simulink model "MMC_Rectifier_NLM_2018"  (R2023b)
settings: Solver=ode23t  StartTime=0.0  StopTime=3  RelTol=1e-3
libraries: spsIGBTDiodeLib x216, spsSeriesRLCBranchLib x117, spsVoltageMeasurementLib x110, spsCurrentMeasurementLib x7, slpidlib x6, spsThreePhaseVIMeasurementLib x2, spsGroundLib x1, spsPower3phInstantaneousLib x1, spsThreePhaseProgrammableVoltageSourceLib x1, spsThreePhaseSeriesRLCBranchLib x1, spspowerguiLib x1
(part 1 of 5)
settings Model: Creator=Administrator  LastModifiedBy=Qu
settings SolverCC: AlgebraicLoopSolver=TrustRegion
settings DataIOCC: ReturnWorkspaceOutputs=off
settings DebuggingCC: ArithmeticOperatorsInVariantConditions=warning
settings SFSimCC: CustomCodeUndefinedFunction=UseInterfaceOnly

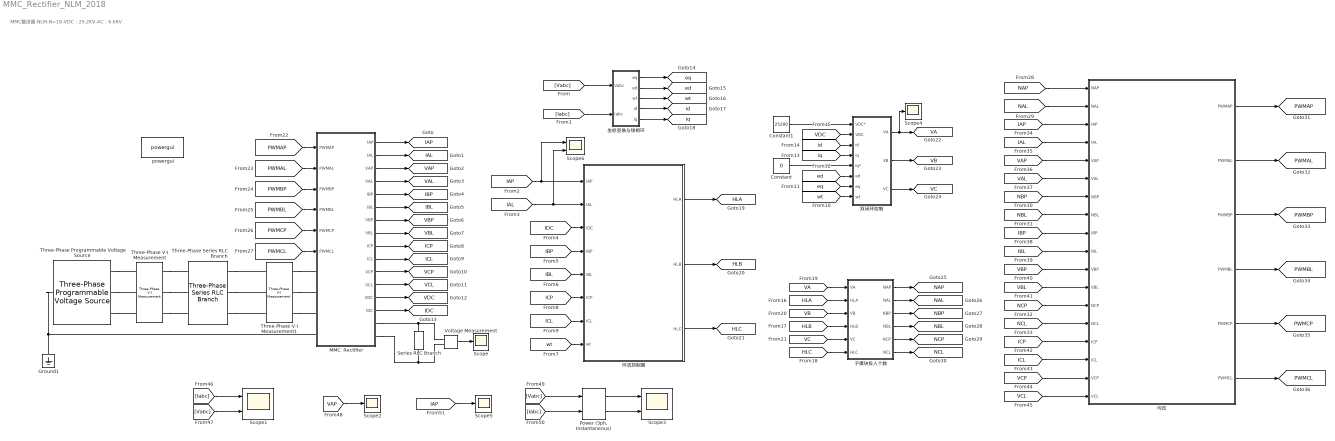
== system MMC_Rectifier_NLM_2018 ==
  note: MMC整流器-NLM-N=18-VDC：25.2KV-AC：6.6KV
  Constant : Constant  Value=0
  Constant1 : Constant  Value=25200
  Ground1 : spsGroundLib/Ground  LConnTagsString=a
  MMC  Rectifier : Subsystem  mask{C0=1.5e-3, V0=1400, C1=1.2e-3, R1=1e-6, L0=0.0577}
      mask prompts: C0 "子模块旁路电容C0"; V0 "子模块电容初始电压V0"; C1 "直流电容C1"; R1 "直流电阻R1"; L0 "桥臂电感L0"
      mask DialogControl ParameterGroupVar Prompt: 参数
  "Power (3ph, Instantaneous)" : spsPower3phInstantaneousLib/Power (3ph, Instantaneous)
  Scope{,2,4..5} (4 alike) : Scope
  Scope1 : Scope  NumInputPorts=2
  Scope3 : Scope  NumInputPorts=2
  Scope6 : Scope  NumInputPorts=2
  Series RLC Branch : spsSeriesRLCBranchLib/Series RLC Branch  LConnTagsString=__new0  RConnTagsString=__new0  BranchType=R  Resistance=200  Inductance=1e-3  SetiL0=off  InitialCurrent=0  Capacitance=1e-6  Setx0=off  InitialVoltage=0  Measurements=None
  Three-Phase Programmable Voltage Source : spsThreePhaseProgrammableVoltageSourceLib/Three-Phase Programmable Voltage Source  PositiveSequence="[6600  0 50]"  VariationEntity=None  VariationType=Table of time-amplitude pairs  VariationTypeAlt=Step  VariationStep=0.5  VariationRate=10  VariationMagnitude=0.3  VariationFrequency=2  VariationTiming=[1 2]  VariationPhaseA=off  Amplitudes=[1 0.8 1.2 1.0]  TimeValues=[0 0.1 0.15 0.2]  HarmonicGeneration=off  HarmonicA=[3 0.2 -25 0]  HarmonicB=[2 0.15 35 2]  Timing="[0.05  3]"  BusType=swing  Pref=0  Qref=0  Qmin=-inf  Qmax=inf
  Three-Phase Series RLC Branch : spsThreePhaseSeriesRLCBranchLib/Three-Phase Series RLC Branch  LConnTagsString=A|B|C  RConnTagsString=A|B|C  BranchType=RL  Resistance=0.5929  Inductance=1e-3  Capacitance=1e-6  Measurements=None
  Three-Phase V-I Measurement : spsThreePhaseVIMeasurementLib/Three-Phase V-I Measurement  VoltageMeasurement=phase-to-ground  SetLabelV=on  LabelV=Vabc  Vpu=off  VpuLL=off  CurrentMeasurement=yes  SetLabelI=on  LabelI=Iabc  Ipu=off  Pbase=100e6  Vbase=500e3  OutputType=Complex  PhasorSimulation=off  PSBequivalent=0
  Three-Phase V-I Measurement1 : spsThreePhaseVIMeasurementLib/Three-Phase V-I Measurement  VoltageMeasurement=phase-to-ground  SetLabelV=on  LabelV=Vin  Vpu=off  VpuLL=off  CurrentMeasurement=yes  SetLabelI=on  LabelI=Iin  Ipu=off  Pbase=100e6  Vbase=500e3  OutputType=Complex  PhasorSimulation=off  PSBequivalent=0
  Voltage Measurement : spsVoltageMeasurementLib/Voltage Measurement  PhasorSimulation=off  OutputType=Complex  PSBequivalent=0
  powergui : spspowerguiLib/powergui  Priority=1  SimulationMode=Discrete  SampleTime=5e-5  frequency=60  Iterations=50  frequencyindice=50  Pbase=100e6  ErrMax=1e-4  UnitsV=kV  UnitsW=MW  buscounter=0  FunctionMessages=off  echomessages=off  EnableUseOfTLC=off  CurrentSourceSwitches=off  DisableSnubberDevices=off  DisableRonSwitches=off  DisableVfSwitches=off  DisplayEquations=off  AutomaticDiscreteSolvers=off  SolverType=Tustin/Backward Euler (TBE)  Interpol=off  ExternalGateDelay=off  methode=off  Ts=100  x0status=blocks  SPID=on  SwTol=0  HookPort=off  NonlinearTolerance=1e-4  nMaxIteration=100  ContinueOnMaxIteration=off  RestoreLinks=warning  ResistiveCurrentMeasurement=off  Frange=[0:2:500]  Ylog=off  Xlog=on  ShowGrid=off  save=off  variable=ZData  structure=0  ZoomFFT=off  StartTime=0.0  cycles=1  DisplayStyle=1  fundamental=60  FreqAxis=off  MaxFrequency=1000  frequencyindicesteady=1  RmsSteady=1  display=off
  双闭环控制 : Subsystem  mask{KP1=0.024467, KI1=0.319, KP2=11.712, KI2=117.263, wL=100*pi*(1e-3+0.0577/2)}
      mask prompts: KP1 "电压外环KP1"; KI1 "电压外环KI1"; KP2 "电流内环KP2"; KI2 "电流内环KI2"; wL "耦合量"
      mask DialogControl ParameterGroupVar Prompt: 参数
  均压 : Subsystem
  坐标变换与锁相环 : Subsystem
  子模块投入个数 : Subsystem  mask{N=18}
      mask prompts: N "子模块个数N"
      mask DialogControl ParameterGroupVar Prompt: 参数
  环流抑制器 : Subsystem  mask{KP=39.04267, KI=117.1793, wL0=100*pi*0.0577}
      mask prompts: KP "环流抑制KP"; KI "环流抑制KI"; wL0 "耦合量wL0"
      mask DialogControl ParameterGroupVar Prompt: 参数
  tag scope: HLA=global, HLB=global, HLC=global, IAL=global, IAP=global, IBL=global, IBP=global, ICL=global, ICP=global, IDC=global, NAL=global, NAP=global, NBL=global, NBP=global, NCL=global, NCP=global, PWMAL=global, PWMAP=global, PWMBL=global, PWMBP=global, PWMCL=global, PWMCP=global, VA=global, VAL=global, VAP=global, VB=global, VBL=global, VBP=global, VC=global, VCL=global, VCP=global, VDC=global, ed=global, eq=global, id=global, iq=global, wt=global
  wires:
  Voltage Measurement/1 -> Scope/1
  MMC  Rectifier/1(IAP) -> [IAP]
  MMC  Rectifier/2(IAL) -> [IAL]
  MMC  Rectifier/3(VAP) -> [VAP]
  MMC  Rectifier/4(VAL) -> [VAL]
  MMC  Rectifier/12(VCL) -> [VCL]
  MMC  Rectifier/11(VCP) -> [VCP]
  MMC  Rectifier/10(ICL) -> [ICL]
  MMC  Rectifier/9(ICP) -> [ICP]
  MMC  Rectifier/8(VBL) -> [VBL]
  MMC  Rectifier/7(VBP) -> [VBP]
  MMC  Rectifier/6(IBL) -> [IBL]
  MMC  Rectifier/5(IBP) -> [IBP]
  MMC  Rectifier/13(VDC) -> [VDC]
  MMC  Rectifier/14(IDC) -> [IDC]
  [Vabc] -> 坐标变换与锁相环/1(Vabc)
  [Iabc] -> 坐标变换与锁相环/2(Iabc)
  坐标变换与锁相环/1(eq) -> [eq]
  坐标变换与锁相环/2(ed) -> [ed]
  坐标变换与锁相环/3(wt) -> [wt]
  坐标变换与锁相环/5(iq) -> [iq]
  坐标变换与锁相环/4(id) -> [id]
  [IAP] -> Scope6/1, 环流抑制器/1(IAP)
  [IAL] -> Scope6/2, 环流抑制器/2(IAL)
  [wt] -> 环流抑制器/8(wt)
  [IDC] -> 环流抑制器/3(IDC)
  [IBP] -> 环流抑制器/4(IBP)
  [IBL] -> 环流抑制器/5(IBL)
  [ICP] -> 环流抑制器/6(ICP)
  [ICL] -> 环流抑制器/7(ICL)
  环流抑制器/2(HLB) -> [HLB]
  环流抑制器/1(HLA) -> [HLA]
  环流抑制器/3(HLC) -> [HLC]
  [wt] -> 双闭环控制/8(wt)
  [eq] -> 双闭环控制/7(eq)
  [ed] -> 双闭环控制/6(ed)
  Constant/1 -> 双闭环控制/5(iq*)
  [id] -> 双闭环控制/3(id)
  [iq] -> 双闭环控制/4(iq)
  [VDC] -> 双闭环控制/2(VDC)
  Constant1/1 -> 双闭环控制/1(VDC*)
  双闭环控制/1(VA) -> Scope4/1, [VA]
  双闭环控制/2(VB) -> [VB]
  双闭环控制/3(VC) -> [VC]
  子模块投入个数/1(NAP) -> [NAP]
  子模块投入个数/2(NAL) -> [NAL]
  子模块投入个数/3(NBP) -> [NBP]
  子模块投入个数/4(NBL) -> [NBL]
  子模块投入个数/5(NCP) -> [NCP]
  子模块投入个数/6(NCL) -> [NCL]
  [HLB] -> 子模块投入个数/4(HLB)
  [HLA] -> 子模块投入个数/2(HLA)
  [HLC] -> 子模块投入个数/6(HLC)
  [VC] -> 子模块投入个数/5(VC)
  [VB] -> 子模块投入个数/3(VB)
  [VA] -> 子模块投入个数/1(VA)
  均压/1(PWMAP) -> [PWMAP]
  均压/2(PWMAL) -> [PWMAL]
  均压/3(PWMBP) -> [PWMBP]
  均压/4(PWMBL) -> [PWMBL]
  均压/5(PWMCP) -> [PWMCP]
  均压/6(PWMCL) -> [PWMCL]
  [PWMBP] -> MMC  Rectifier/3(PWMBP)
  [PWMBL] -> MMC  Rectifier/4(PWMBL)
  [PWMAL] -> MMC  Rectifier/2(PWMAL)
  [PWMAP] -> MMC  Rectifier/1(PWMAP)
  [PWMCP] -> MMC  Rectifier/5(PWMCP)
  [PWMCL] -> MMC  Rectifier/6(PWMCL)
  [NAP] -> 均压/1(NAP)
  [NAL] -> 均压/2(NAL)
  [NBP] -> 均压/7(NBP)
  [NBL] -> 均压/8(NBL)
  [NCP] -> 均压/13(NCP)
  [NCL] -> 均压/14(NCL)
  [IAP] -> 均压/3(IAP)
  [IAL] -> 均压/4(IAL)
  [VAL] -> 均压/6(VAL)
  [VAP] -> 均压/5(VAP)
  [IBP] -> 均压/9(IBP)
  [IBL] -> 均压/10(IBL)
  [VBP] -> 均压/11(VBP)
  [VBL] -> 均压/12(VBL)
  [VCP] -> 均压/17(VCP)
  [ICL] -> 均压/16(ICL)
  [ICP] -> 均压/15(ICP)
  [VCL] -> 均压/18(VCL)
  [Iabc] -> Scope1/1
  [Vabc] -> Scope1/2
  [VAP] -> Scope2/1
  [Vabc] -> "Power (3ph, Instantaneous)"/1
  [Iabc] -> "Power (3ph, Instantaneous)"/2
  "Power (3ph, Instantaneous)"/1 -> Scope3/1
  "Power (3ph, Instantaneous)"/2 -> Scope3/2
  [IAP] -> Scope5/1
  connections:
  Three-Phase Programmable Voltage Source/LConn1 -- MMC  Rectifier/LConn4 -- Ground1/LConn1
  Three-Phase Programmable Voltage Source/RConn1 -- Three-Phase V-I Measurement/LConn1
  Three-Phase Programmable Voltage Source/RConn2 -- Three-Phase V-I Measurement/LConn2
  Three-Phase Programmable Voltage Source/RConn3 -- Three-Phase V-I Measurement/LConn3
  Three-Phase V-I Measurement/RConn1 -- Three-Phase Series RLC Branch/LConn1
  Three-Phase V-I Measurement/RConn2 -- Three-Phase Series RLC Branch/LConn2
  Three-Phase V-I Measurement/RConn3 -- Three-Phase Series RLC Branch/LConn3
  Three-Phase Series RLC Branch/RConn1 -- Three-Phase V-I Measurement1/LConn1
  Three-Phase Series RLC Branch/RConn2 -- Three-Phase V-I Measurement1/LConn2
  Three-Phase Series RLC Branch/RConn3 -- Three-Phase V-I Measurement1/LConn3
  Three-Phase V-I Measurement1/RConn1 -- MMC  Rectifier/LConn1
  Three-Phase V-I Measurement1/RConn2 -- MMC  Rectifier/LConn2
  Three-Phase V-I Measurement1/RConn3 -- MMC  Rectifier/LConn3
  MMC  Rectifier/RConn1 -- Voltage Measurement/LConn1 -- Series RLC Branch/LConn1
  MMC  Rectifier/RConn2 -- Voltage Measurement/LConn2 -- Series RLC Branch/RConn1

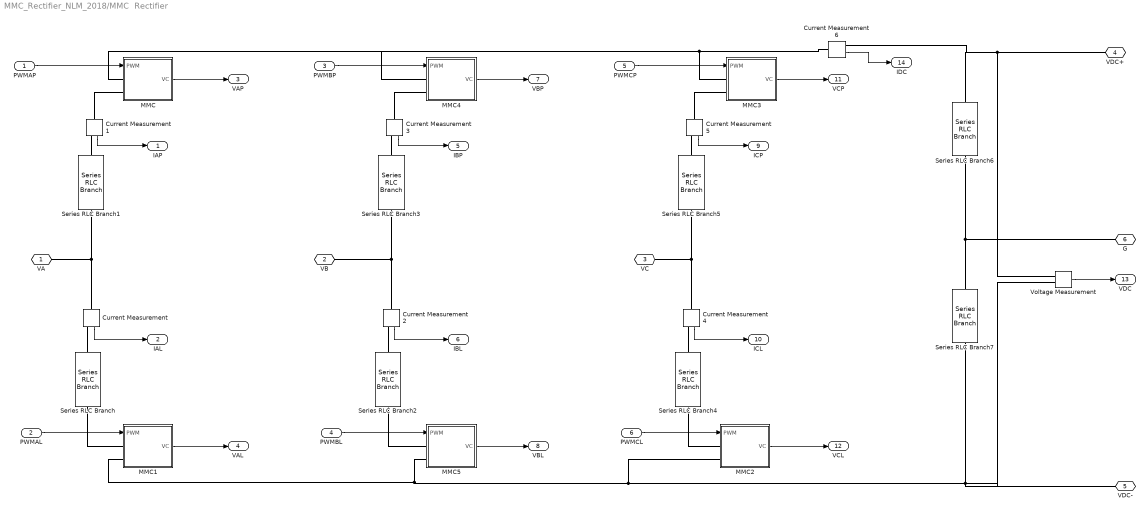
== system MMC_Rectifier_NLM_2018/MMC  Rectifier ==
  PWMAP : Inport
  PWMAL : Inport  Port=2
  PWMBP : Inport  Port=3
  PWMBL : Inport  Port=4
  PWMCP : Inport  Port=5
  PWMCL : Inport  Port=6
  Current Measurement{,1..6} (7 alike) : spsCurrentMeasurementLib/Current Measurement  PhasorSimulation=off  OutputType=Complex  PSBequivalent=0
  MMC : Subsystem
  MMC1 : Subsystem
  MMC2 : Subsystem
  MMC3 : Subsystem
  MMC4 : Subsystem
  MMC5 : Subsystem
  Series RLC Branch{,1..5} (6 alike) : spsSeriesRLCBranchLib/Series RLC Branch  LConnTagsString=__new0  RConnTagsString=__new0  BranchType=L  Resistance=1  Inductance=L0  SetiL0=off  InitialCurrent=0  Capacitance=1e-6  Setx0=off  InitialVoltage=0  Measurements=None
  Series RLC Branch6 : spsSeriesRLCBranchLib/Series RLC Branch  LConnTagsString=__new0  RConnTagsString=__new0  BranchType=RC  Resistance=R1  Inductance=L0  SetiL0=off  InitialCurrent=0  Capacitance=2*C1  Setx0=off  InitialVoltage=3000  Measurements=None
  Series RLC Branch7 : spsSeriesRLCBranchLib/Series RLC Branch  LConnTagsString=__new0  RConnTagsString=__new0  BranchType=RC  Resistance=R1  Inductance=L0  SetiL0=off  InitialCurrent=0  Capacitance=2*C1  Setx0=off  InitialVoltage=3000  Measurements=None
  Voltage Measurement : spsVoltageMeasurementLib/Voltage Measurement  PhasorSimulation=off  OutputType=Complex  PSBequivalent=0
  VA : PMIOPort  Side=Left
  VB : PMIOPort  Port=2  Side=Left
  VC : PMIOPort  Port=3  Side=Left
  VDC+ : PMIOPort  Port=4  Side=Right
  VDC- : PMIOPort  Port=5  Side=Right
  G : PMIOPort  Port=6  Side=Left
  IAP : Outport
  IAL : Outport  Port=2
  VAP : Outport  Port=3
  VAL : Outport  Port=4
  IBP : Outport  Port=5
  IBL : Outport  Port=6
  VBP : Outport  Port=7
  VBL : Outport  Port=8
  ICP : Outport  Port=9
  ICL : Outport  Port=10
  VCP : Outport  Port=11
  VCL : Outport  Port=12
  VDC : Outport  Port=13
  IDC : Outport  Port=14
  wires:
  MMC4/1(VC) -> VBP/1
  Current Measurement1/1 -> IAP/1
  Voltage Measurement/1 -> VDC/1
  PWMAL/1 -> MMC1/1(PWM)
  MMC2/1(VC) -> VCL/1
  MMC/1(VC) -> VAP/1
  MMC1/1(VC) -> VAL/1
  Current Measurement/1 -> IAL/1
  Current Measurement4/1 -> ICL/1
  MMC3/1(VC) -> VCP/1
  MMC5/1(VC) -> VBL/1
  PWMBL/1 -> MMC5/1(PWM)
  PWMBP/1 -> MMC4/1(PWM)
  Current Measurement2/1 -> IBL/1
  Current Measurement3/1 -> IBP/1
  PWMAP/1 -> MMC/1(PWM)
  Current Measurement5/1 -> ICP/1
  PWMCP/1 -> MMC3/1(PWM)
  PWMCL/1 -> MMC2/1(PWM)
  Current Measurement6/1 -> IDC/1
  connections:
  MMC5/LConn1 -- Series RLC Branch2/RConn1
  Series RLC Branch3/RConn1 -- VB/RConn1 -- Current Measurement2/LConn1
  Current Measurement2/RConn1 -- Series RLC Branch2/LConn1
  VDC+/RConn1 -- Current Measurement6/RConn1 -- Series RLC Branch6/LConn1 -- Voltage Measurement/LConn1
  MMC1/LConn1 -- Series RLC Branch/RConn1
  VDC-/RConn1 -- Voltage Measurement/LConn2 -- Series RLC Branch7/RConn1 -- MMC2/LConn2 -- MMC5/LConn2 -- MMC1/LConn2
  Current Measurement3/RConn1 -- Series RLC Branch3/LConn1
  Series RLC Branch5/RConn1 -- VC/RConn1 -- Current Measurement4/LConn1
  Current Measurement5/RConn1 -- Series RLC Branch5/LConn1
  Series RLC Branch1/RConn1 -- VA/RConn1 -- Current Measurement/LConn1
  Current Measurement/RConn1 -- Series RLC Branch/LConn1
  MMC/LConn2 -- Current Measurement1/LConn1
  Current Measurement1/RConn1 -- Series RLC Branch1/LConn1
  MMC4/LConn2 -- Current Measurement3/LConn1
  Current Measurement4/RConn1 -- Series RLC Branch4/LConn1
  MMC2/LConn1 -- Series RLC Branch4/RConn1
  Series RLC Branch6/RConn1 -- G/RConn1 -- Series RLC Branch7/LConn1
  MMC4/LConn1 -- MMC/LConn1 -- MMC3/LConn1 -- Current Measurement6/LConn1
  MMC3/LConn2 -- Current Measurement5/LConn1

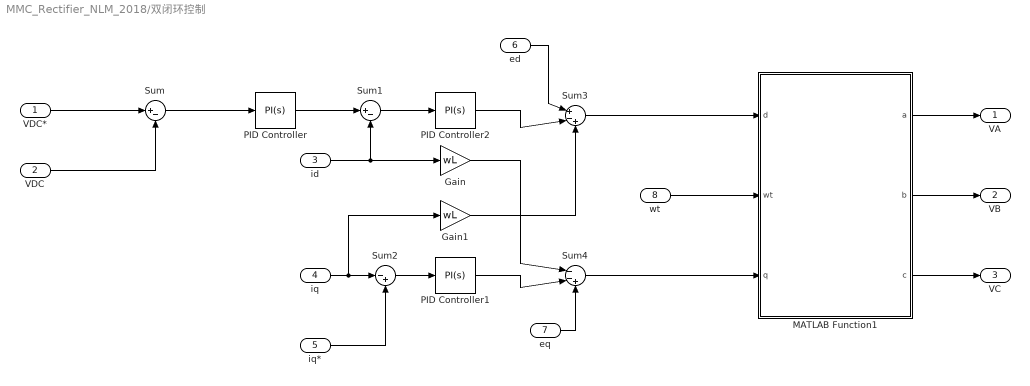
== system MMC_Rectifier_NLM_2018/双闭环控制 ==
  VDC* : Inport
  VDC : Inport  Port=2
  id : Inport  Port=3
  iq : Inport  Port=4
  iq* : Inport  Port=5
  ed : Inport  Port=6
  eq : Inport  Port=7
  wt : Inport  Port=8
  Gain : Gain  Gain=wL
  Gain1 : Gain  Gain=wL
  MATLAB Function1 : MATLAB Function  TreatAsAtomicUnit=on
  PID Controller : slpidlib/PID Controller  Controller=PI  Form=Parallel  TimeDomain=Continuous-time  UseExternalTs=off  SampleTime=-1  IntegratorMethod=Forward Euler  FilterMethod=Forward Euler  ControllerParametersSource=internal  P=KP1  I=KI1  UseKiTs=off  D=0  N=100  UseFilter=on  TunerSelectOption=Transfer Function Based (PID Tuner App)  InitialConditionSource=internal  InitialConditionForIntegrator=0  InitialConditionForFilter=0  DifferentiatorICPrevScaledInput=0  ExternalReset=none  TrackingMode=off  Kt=1  LimitOutput=off  SatLimitsSource=internal  UpperSaturationLimit=inf  LowerSaturationLimit=-inf  LinearizeAsGain=on  AntiWindupMode=none  Kb=1  LimitIntegrator=off  UpperIntegratorSaturationLimit=inf  LowerIntegratorSaturationLimit=-inf  POutMin=[]  POutMax=[]  IOutMin=[]  IOutMax=[]  DOutMin=[]  DOutMax=[]  NOutMin=[]  NOutMax=[]  SumOutMin=[]  SumOutMax=[]  SaturationOutMin=[]  SaturationOutMax=[]  PParamMin=[]  PParamMax=[]  IParamMin=[]  IParamMax=[]  DParamMin=[]  DParamMax=[]  NParamMin=[]  NParamMax=[]  KbParamMin=[]  KbParamMax=[]  KtParamMin=[]  KtParamMax=[]  KbOutMin=[]  KbOutMax=[]  KtOutMin=[]  KtOutMax=[]  IntegratorOutMin=[]  IntegratorOutMax=[]  FilterOutMin=[]  FilterOutMax=[]  SumI1OutMin=[]  SumI1OutMax=[]  SumI2OutMin=[]  SumI2OutMax=[]  SumI3OutMin=[]  SumI3OutMax=[]  SumI4OutMin=[]  SumI4OutMax=[]  SumDOutMin=[]  SumDOutMax=[]  DifferentiatorOutMin=[]  DifferentiatorOutMax=[]  FilterDiffOutCoefMin=[]  FilterDiffOutCoefMax=[]  ReciprocalOutMin=[]  ReciprocalOutMax=[]  SumDenOutMin=[]  SumDenOutMax=[]  SumNumOutMin=[]  SumNumOutMax=[]  DivideOutMin=[]  DivideOutMax=[]  UdiffTsProdOutMin=[]  UdiffTsProdOutMax=[]  NTsProdOutMin=[]  NTsProdOutMax=[]  UintegralTsProdOutMin=[]  UintegralTsProdOutMax=[]  UngainTsProdOutMin=[]  UngainTsProdOutMax=[]  ClampingZeroOutDataTypeStr=Inherit: Inherit via back propagation  ClampingZeroOutMin=[]  ClampingZeroOutMax=[]  FilterDenConstantOutDataTypeStr=Inherit: Inherit via back propagation  FilterDenConstantOutMin=[]  FilterDenConstantOutMax=[]  PCopyOutDataTypeStr=Inherit: Inherit via back propagation  PCopyOutMin=[]  PCopyOutMax=[]  NCopyOutDataTypeStr=Inherit: Inherit via back propagation  NCopyOutMin=[]  NCopyOutMax=[]  IntegratorContinuousStateAttributes=''  IntegratorStateMustResolveToSignalObject=off  IntegratorRTWStateStorageClass=Auto  FilterContinuousStateAttributes=''  FilterStateMustResolveToSignalObject=off  FilterRTWStateStorageClass=Auto  ParallelPVariant=InternalParameters  IdealPVariant=Disabled  IVariant=InternalParameters  DVariant=Disabled  IntegratorVariant=Continuous  SatVariant=Disabled  AWVariant=Passthrough  PCopyVariant=Disabled  TRVariant=Disabled  FdbkBlocksVariant=Forward  IdealPFdbkVariant=Disabled  SatFdbkVariant=Disabled  DerivativeFilterVariant=Disabled  NVariant=Disabled  NCopyVariant=Disabled_SignalSpec  FilterICVariant=Disabled  IntegratorICVariant=InternalICs  ExternalResetVariant=Disabled  TRSumVariant=Passthrough  SumFdbkVariant=Disabled  SumVariant=Sum_PI  TsampFilterVariant=InternalTs  TsampNgainVariant=Passthrough  TsampIntegralVariant=Disabled_SignalSpec  ExternalSaturationOutDataTypeStr=Inherit: Same as second input
  PID Controller1 : slpidlib/PID Controller  Controller=PI  Form=Parallel  TimeDomain=Continuous-time  UseExternalTs=off  SampleTime=-1  IntegratorMethod=Forward Euler  FilterMethod=Forward Euler  ControllerParametersSource=internal  P=KP2  I=KI2  UseKiTs=off  D=0  N=100  UseFilter=on  TunerSelectOption=Transfer Function Based (PID Tuner App)  InitialConditionSource=internal  InitialConditionForIntegrator=0  InitialConditionForFilter=0  DifferentiatorICPrevScaledInput=0  ExternalReset=none  TrackingMode=off  Kt=1  LimitOutput=off  SatLimitsSource=internal  UpperSaturationLimit=inf  LowerSaturationLimit=-inf  LinearizeAsGain=on  AntiWindupMode=none  Kb=1  LimitIntegrator=off  UpperIntegratorSaturationLimit=inf  LowerIntegratorSaturationLimit=-inf  POutMin=[]  POutMax=[]  IOutMin=[]  IOutMax=[]  DOutMin=[]  DOutMax=[]  NOutMin=[]  NOutMax=[]  SumOutMin=[]  SumOutMax=[]  SaturationOutMin=[]  SaturationOutMax=[]  PParamMin=[]  PParamMax=[]  IParamMin=[]  IParamMax=[]  DParamMin=[]  DParamMax=[]  NParamMin=[]  NParamMax=[]  KbParamMin=[]  KbParamMax=[]  KtParamMin=[]  KtParamMax=[]  KbOutMin=[]  KbOutMax=[]  KtOutMin=[]  KtOutMax=[]  IntegratorOutMin=[]  IntegratorOutMax=[]  FilterOutMin=[]  FilterOutMax=[]  SumI1OutMin=[]  SumI1OutMax=[]  SumI2OutMin=[]  SumI2OutMax=[]  SumI3OutMin=[]  SumI3OutMax=[]  SumI4OutMin=[]  SumI4OutMax=[]  SumDOutMin=[]  SumDOutMax=[]  DifferentiatorOutMin=[]  DifferentiatorOutMax=[]  FilterDiffOutCoefMin=[]  FilterDiffOutCoefMax=[]  ReciprocalOutMin=[]  ReciprocalOutMax=[]  SumDenOutMin=[]  SumDenOutMax=[]  SumNumOutMin=[]  SumNumOutMax=[]  DivideOutMin=[]  DivideOutMax=[]  UdiffTsProdOutMin=[]  UdiffTsProdOutMax=[]  NTsProdOutMin=[]  NTsProdOutMax=[]  UintegralTsProdOutMin=[]  UintegralTsProdOutMax=[]  UngainTsProdOutMin=[]  UngainTsProdOutMax=[]  ClampingZeroOutDataTypeStr=Inherit: Inherit via back propagation  ClampingZeroOutMin=[]  ClampingZeroOutMax=[]  FilterDenConstantOutDataTypeStr=Inherit: Inherit via back propagation  FilterDenConstantOutMin=[]  FilterDenConstantOutMax=[]  PCopyOutDataTypeStr=Inherit: Inherit via back propagation  PCopyOutMin=[]  PCopyOutMax=[]  NCopyOutDataTypeStr=Inherit: Inherit via back propagation  NCopyOutMin=[]  NCopyOutMax=[]  IntegratorContinuousStateAttributes=''  IntegratorStateMustResolveToSignalObject=off  IntegratorRTWStateStorageClass=Auto  FilterContinuousStateAttributes=''  FilterStateMustResolveToSignalObject=off  FilterRTWStateStorageClass=Auto  ParallelPVariant=InternalParameters  IdealPVariant=Disabled  IVariant=InternalParameters  DVariant=Disabled  IntegratorVariant=Continuous  SatVariant=Disabled  AWVariant=Passthrough  PCopyVariant=Disabled  TRVariant=Disabled  FdbkBlocksVariant=Forward  IdealPFdbkVariant=Disabled  SatFdbkVariant=Disabled  DerivativeFilterVariant=Disabled  NVariant=Disabled  NCopyVariant=Disabled_SignalSpec  FilterICVariant=Disabled  IntegratorICVariant=InternalICs  ExternalResetVariant=Disabled  TRSumVariant=Passthrough  SumFdbkVariant=Disabled  SumVariant=Sum_PI  TsampFilterVariant=InternalTs  TsampNgainVariant=Passthrough  TsampIntegralVariant=Disabled_SignalSpec  ExternalSaturationOutDataTypeStr=Inherit: Same as second input
  PID Controller2 : slpidlib/PID Controller  Controller=PI  Form=Parallel  TimeDomain=Continuous-time  UseExternalTs=off  SampleTime=-1  IntegratorMethod=Forward Euler  FilterMethod=Forward Euler  ControllerParametersSource=internal  P=KP2  I=KI2  UseKiTs=off  D=0  N=100  UseFilter=on  TunerSelectOption=Transfer Function Based (PID Tuner App)  InitialConditionSource=internal  InitialConditionForIntegrator=0  InitialConditionForFilter=0  DifferentiatorICPrevScaledInput=0  ExternalReset=none  TrackingMode=off  Kt=1  LimitOutput=off  SatLimitsSource=internal  UpperSaturationLimit=inf  LowerSaturationLimit=-inf  LinearizeAsGain=on  AntiWindupMode=none  Kb=1  LimitIntegrator=off  UpperIntegratorSaturationLimit=inf  LowerIntegratorSaturationLimit=-inf  POutMin=[]  POutMax=[]  IOutMin=[]  IOutMax=[]  DOutMin=[]  DOutMax=[]  NOutMin=[]  NOutMax=[]  SumOutMin=[]  SumOutMax=[]  SaturationOutMin=[]  SaturationOutMax=[]  PParamMin=[]  PParamMax=[]  IParamMin=[]  IParamMax=[]  DParamMin=[]  DParamMax=[]  NParamMin=[]  NParamMax=[]  KbParamMin=[]  KbParamMax=[]  KtParamMin=[]  KtParamMax=[]  KbOutMin=[]  KbOutMax=[]  KtOutMin=[]  KtOutMax=[]  IntegratorOutMin=[]  IntegratorOutMax=[]  FilterOutMin=[]  FilterOutMax=[]  SumI1OutMin=[]  SumI1OutMax=[]  SumI2OutMin=[]  SumI2OutMax=[]  SumI3OutMin=[]  SumI3OutMax=[]  SumI4OutMin=[]  SumI4OutMax=[]  SumDOutMin=[]  SumDOutMax=[]  DifferentiatorOutMin=[]  DifferentiatorOutMax=[]  FilterDiffOutCoefMin=[]  FilterDiffOutCoefMax=[]  ReciprocalOutMin=[]  ReciprocalOutMax=[]  SumDenOutMin=[]  SumDenOutMax=[]  SumNumOutMin=[]  SumNumOutMax=[]  DivideOutMin=[]  DivideOutMax=[]  UdiffTsProdOutMin=[]  UdiffTsProdOutMax=[]  NTsProdOutMin=[]  NTsProdOutMax=[]  UintegralTsProdOutMin=[]  UintegralTsProdOutMax=[]  UngainTsProdOutMin=[]  UngainTsProdOutMax=[]  ClampingZeroOutDataTypeStr=Inherit: Inherit via back propagation  ClampingZeroOutMin=[]  ClampingZeroOutMax=[]  FilterDenConstantOutDataTypeStr=Inherit: Inherit via back propagation  FilterDenConstantOutMin=[]  FilterDenConstantOutMax=[]  PCopyOutDataTypeStr=Inherit: Inherit via back propagation  PCopyOutMin=[]  PCopyOutMax=[]  NCopyOutDataTypeStr=Inherit: Inherit via back propagation  NCopyOutMin=[]  NCopyOutMax=[]  IntegratorContinuousStateAttributes=''  IntegratorStateMustResolveToSignalObject=off  IntegratorRTWStateStorageClass=Auto  FilterContinuousStateAttributes=''  FilterStateMustResolveToSignalObject=off  FilterRTWStateStorageClass=Auto  ParallelPVariant=InternalParameters  IdealPVariant=Disabled  IVariant=InternalParameters  DVariant=Disabled  IntegratorVariant=Continuous  SatVariant=Disabled  AWVariant=Passthrough  PCopyVariant=Disabled  TRVariant=Disabled  FdbkBlocksVariant=Forward  IdealPFdbkVariant=Disabled  SatFdbkVariant=Disabled  DerivativeFilterVariant=Disabled  NVariant=Disabled  NCopyVariant=Disabled_SignalSpec  FilterICVariant=Disabled  IntegratorICVariant=InternalICs  ExternalResetVariant=Disabled  TRSumVariant=Passthrough  SumFdbkVariant=Disabled  SumVariant=Sum_PI  TsampFilterVariant=InternalTs  TsampNgainVariant=Passthrough  TsampIntegralVariant=Disabled_SignalSpec  ExternalSaturationOutDataTypeStr=Inherit: Same as second input
  Sum : Sum  Inputs=|+-
  Sum1 : Sum  Inputs=|+-
  Sum2 : Sum  Inputs=|-+
  Sum3 : Sum  Inputs=|+-+
  Sum4 : Sum  Inputs=|--+
  VA : Outport
  VB : Outport  Port=2
  VC : Outport  Port=3
  wires:
  ed/1 -> Sum3/1
  iq*/1 -> Sum2/2
  VDC*/1 -> Sum/1
  VDC/1 -> Sum/2
  iq/1 -> Gain1/1, Sum2/1
  Sum3/1 -> MATLAB Function1/1(d)
  Sum4/1 -> MATLAB Function1/3(q)
  PID Controller1/1 -> Sum4/2
  Sum2/1 -> PID Controller1/1
  MATLAB Function1/1(a) -> VA/1
  id/1 -> Gain/1, Sum1/2
  Sum/1 -> PID Controller/1
  Sum1/1 -> PID Controller2/1
  PID Controller/1 -> Sum1/1
  Gain1/1 -> Sum3/3
  wt/1 -> MATLAB Function1/2(wt)
  MATLAB Function1/3(c) -> VC/1
  PID Controller2/1 -> Sum3/2
  MATLAB Function1/2(b) -> VB/1
  Gain/1 -> Sum4/1
  eq/1 -> Sum4/3

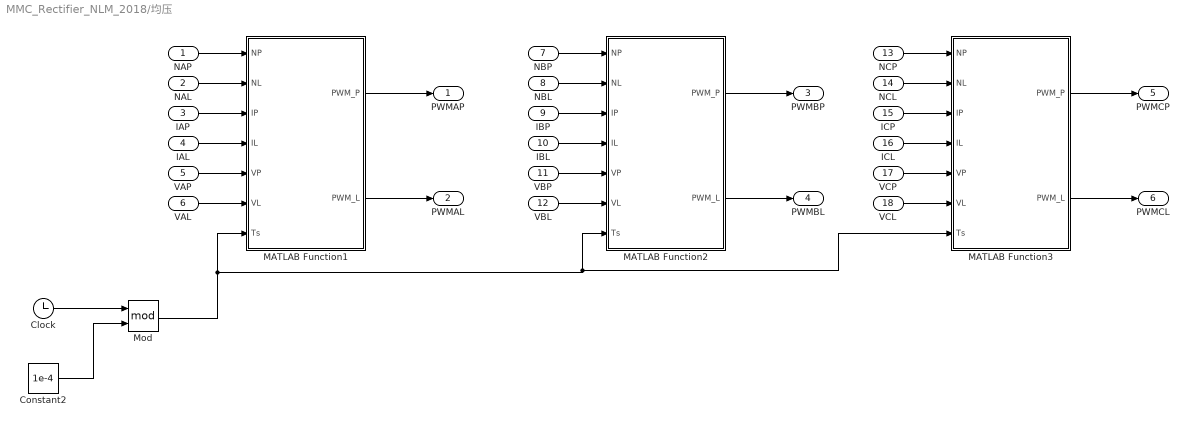
== system MMC_Rectifier_NLM_2018/均压 ==
  NAP : Inport
  NAL : Inport  Port=2
  IAP : Inport  Port=3
  IAL : Inport  Port=4
  VAP : Inport  Port=5
  VAL : Inport  Port=6
  NBP : Inport  Port=7
  NBL : Inport  Port=8
  IBP : Inport  Port=9
  IBL : Inport  Port=10
  VBP : Inport  Port=11
  VBL : Inport  Port=12
  NCP : Inport  Port=13
  NCL : Inport  Port=14
  ICP : Inport  Port=15
  ICL : Inport  Port=16
  VCP : Inport  Port=17
  VCL : Inport  Port=18
  Clock : Clock
  Constant2 : Constant  Value=1e-4
  MATLAB Function1 : MATLAB Function  TreatAsAtomicUnit=on
  MATLAB Function2 : MATLAB Function  TreatAsAtomicUnit=on
  MATLAB Function3 : MATLAB Function  TreatAsAtomicUnit=on
  Mod : Math  Operator=mod  SignedPower=on
  PWMAP : Outport
  PWMAL : Outport  Port=2
  PWMBP : Outport  Port=3
  PWMBL : Outport  Port=4
  PWMCP : Outport  Port=5
  PWMCL : Outport  Port=6
  wires:
  NAL/1 -> MATLAB Function1/2(NL)
  NCP/1 -> MATLAB Function3/1(NP)
  Constant2/1 -> Mod/2
  Mod/1 -> MATLAB Function1/7(Ts), MATLAB Function3/7(Ts), MATLAB Function2/7(Ts)
  VCP/1 -> MATLAB Function3/5(VP)
  MATLAB Function2/2(PWM_L) -> PWMBL/1
  IAP/1 -> MATLAB Function1/3(IP)
  Clock/1 -> Mod/1
  MATLAB Function1/2(PWM_L) -> PWMAL/1
  ICL/1 -> MATLAB Function3/4(IL)
  MATLAB Function1/1(PWM_P) -> PWMAP/1
  VBL/1 -> MATLAB Function2/6(VL)
  IAL/1 -> MATLAB Function1/4(IL)
  MATLAB Function3/2(PWM_L) -> PWMCL/1
  VBP/1 -> MATLAB Function2/5(VP)
  VAL/1 -> MATLAB Function1/6(VL)
  VCL/1 -> MATLAB Function3/6(VL)
  MATLAB Function2/1(PWM_P) -> PWMBP/1
  NBP/1 -> MATLAB Function2/1(NP)
  NBL/1 -> MATLAB Function2/2(NL)
  ICP/1 -> MATLAB Function3/3(IP)
  IBP/1 -> MATLAB Function2/3(IP)
  IBL/1 -> MATLAB Function2/4(IL)
  NAP/1 -> MATLAB Function1/1(NP)
  VAP/1 -> MATLAB Function1/5(VP)
  MATLAB Function3/1(PWM_P) -> PWMCP/1
  NCL/1 -> MATLAB Function3/2(NL)

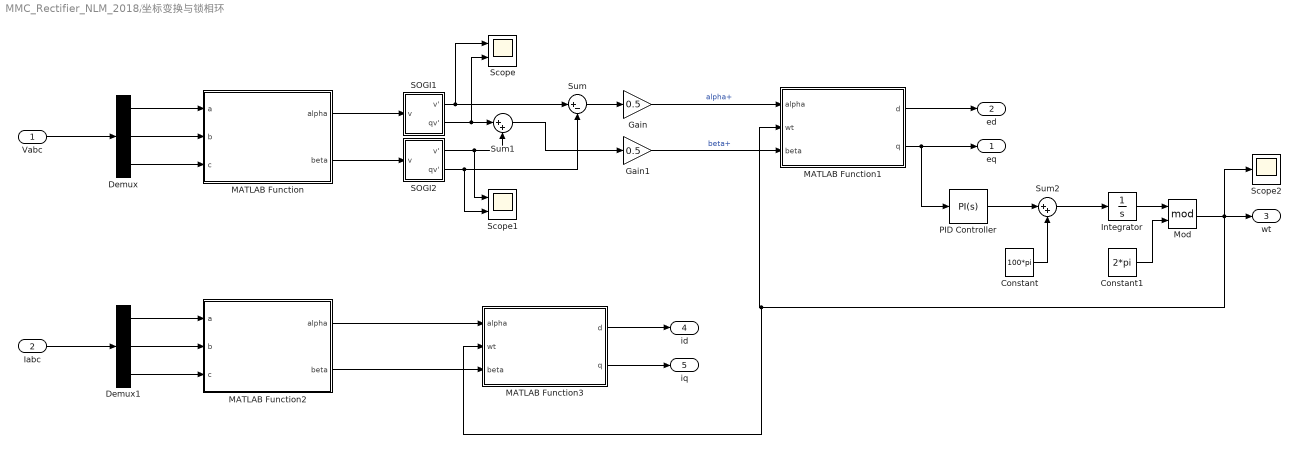
== system MMC_Rectifier_NLM_2018/坐标变换与锁相环 ==
  Vabc : Inport
  Iabc : Inport  Port=2
  Constant : Constant  Value=100*pi
  Constant1 : Constant  Value=2*pi
  Demux : Demux  Outputs=3
  Demux1 : Demux  Outputs=3
  Gain : Gain  Gain=0.5
  Gain1 : Gain  Gain=0.5
  Integrator : Integrator
  MATLAB Function : MATLAB Function  TreatAsAtomicUnit=on
  MATLAB Function1 : MATLAB Function  TreatAsAtomicUnit=on
  MATLAB Function2 : MATLAB Function  TreatAsAtomicUnit=on
  MATLAB Function3 : MATLAB Function  TreatAsAtomicUnit=on
  Mod : Math  Operator=mod  SignedPower=on
  PID Controller : slpidlib/PID Controller  Controller=PI  Form=Parallel  TimeDomain=Continuous-time  UseExternalTs=off  SampleTime=-1  IntegratorMethod=Forward Euler  FilterMethod=Forward Euler  ControllerParametersSource=internal  P=5  I=1/200  UseKiTs=off  D=0  N=100  UseFilter=on  TunerSelectOption=Transfer Function Based (PID Tuner App)  InitialConditionSource=internal  InitialConditionForIntegrator=0  InitialConditionForFilter=0  DifferentiatorICPrevScaledInput=0  ExternalReset=none  TrackingMode=off  Kt=1  LimitOutput=off  SatLimitsSource=internal  UpperSaturationLimit=inf  LowerSaturationLimit=-inf  LinearizeAsGain=on  AntiWindupMode=none  Kb=1  LimitIntegrator=off  UpperIntegratorSaturationLimit=inf  LowerIntegratorSaturationLimit=-inf  POutMin=[]  POutMax=[]  IOutMin=[]  IOutMax=[]  DOutMin=[]  DOutMax=[]  NOutMin=[]  NOutMax=[]  SumOutMin=[]  SumOutMax=[]  SaturationOutMin=[]  SaturationOutMax=[]  PParamMin=[]  PParamMax=[]  IParamMin=[]  IParamMax=[]  DParamMin=[]  DParamMax=[]  NParamMin=[]  NParamMax=[]  KbParamMin=[]  KbParamMax=[]  KtParamMin=[]  KtParamMax=[]  KbOutMin=[]  KbOutMax=[]  KtOutMin=[]  KtOutMax=[]  IntegratorOutMin=[]  IntegratorOutMax=[]  FilterOutMin=[]  FilterOutMax=[]  SumI1OutMin=[]  SumI1OutMax=[]  SumI2OutMin=[]  SumI2OutMax=[]  SumI3OutMin=[]  SumI3OutMax=[]  SumI4OutMin=[]  SumI4OutMax=[]  SumDOutMin=[]  SumDOutMax=[]  DifferentiatorOutMin=[]  DifferentiatorOutMax=[]  FilterDiffOutCoefMin=[]  FilterDiffOutCoefMax=[]  ReciprocalOutMin=[]  ReciprocalOutMax=[]  SumDenOutMin=[]  SumDenOutMax=[]  SumNumOutMin=[]  SumNumOutMax=[]  DivideOutMin=[]  DivideOutMax=[]  UdiffTsProdOutMin=[]  UdiffTsProdOutMax=[]  NTsProdOutMin=[]  NTsProdOutMax=[]  UintegralTsProdOutMin=[]  UintegralTsProdOutMax=[]  UngainTsProdOutMin=[]  UngainTsProdOutMax=[]  ClampingZeroOutDataTypeStr=Inherit: Inherit via back propagation  ClampingZeroOutMin=[]  ClampingZeroOutMax=[]  FilterDenConstantOutDataTypeStr=Inherit: Inherit via back propagation  FilterDenConstantOutMin=[]  FilterDenConstantOutMax=[]  PCopyOutDataTypeStr=Inherit: Inherit via back propagation  PCopyOutMin=[]  PCopyOutMax=[]  NCopyOutDataTypeStr=Inherit: Inherit via back propagation  NCopyOutMin=[]  NCopyOutMax=[]  IntegratorContinuousStateAttributes=''  IntegratorStateMustResolveToSignalObject=off  IntegratorRTWStateStorageClass=Auto  FilterContinuousStateAttributes=''  FilterStateMustResolveToSignalObject=off  FilterRTWStateStorageClass=Auto  ParallelPVariant=InternalParameters  IdealPVariant=Disabled  IVariant=InternalParameters  DVariant=Disabled  IntegratorVariant=Continuous  SatVariant=Disabled  AWVariant=Passthrough  PCopyVariant=Disabled  TRVariant=Disabled  FdbkBlocksVariant=Forward  IdealPFdbkVariant=Disabled  SatFdbkVariant=Disabled  DerivativeFilterVariant=Disabled  NVariant=Disabled  NCopyVariant=Disabled_SignalSpec  FilterICVariant=Disabled  IntegratorICVariant=InternalICs  ExternalResetVariant=Disabled  TRSumVariant=Passthrough  SumFdbkVariant=Disabled  SumVariant=Sum_PI  TsampFilterVariant=InternalTs  TsampNgainVariant=Passthrough  TsampIntegralVariant=Disabled_SignalSpec  ExternalSaturationOutDataTypeStr=Inherit: Same as second input
  SOGI1 : Subsystem
  SOGI2 : Subsystem
  Scope : Scope  NumInputPorts=2
  Scope1 : Scope  NumInputPorts=2
  Scope2 : Scope
  Sum : Sum  Inputs=|+-
  Sum1 : Sum  Inputs=|++
  Sum2 : Sum  Inputs=|++
  eq : Outport
  ed : Outport  Port=2
  wt : Outport  Port=3
  id : Outport  Port=4
  iq : Outport  Port=5
  wires:
  Demux/3 -> MATLAB Function/3(c)
  MATLAB Function1/2(q) -> PID Controller/1, eq/1
  Gain/1 -> MATLAB Function1/1(alpha)  "alpha+"
  Vabc/1 -> Demux/1
  Gain1/1 -> MATLAB Function1/3(beta)  "beta+"
  Demux/2 -> MATLAB Function/2(b)
  Demux/1 -> MATLAB Function/1(a)
  SOGI2/2(qv') -> Scope1/2, Sum/2
  Iabc/1 -> Demux1/1
  Sum1/1 -> Gain1/1
  Demux1/2 -> MATLAB Function2/2(b)
  MATLAB Function/2(beta) -> SOGI2/1(v)
  MATLAB Function2/2(beta) -> MATLAB Function3/3(beta)
  SOGI1/1(v') -> Scope/1, Sum/1
  MATLAB Function/1(alpha) -> SOGI1/1(v)
  SOGI1/2(qv') -> Scope/2, Sum1/1
  Sum/1 -> Gain/1
  SOGI2/1(v') -> Scope1/1, Sum1/2
  MATLAB Function1/1(d) -> ed/1
  Constant/1 -> Sum2/2
  MATLAB Function3/2(q) -> iq/1
  PID Controller/1 -> Sum2/1
  Integrator/1 -> Mod/1
  Demux1/1 -> MATLAB Function2/1(a)
  Demux1/3 -> MATLAB Function2/3(c)
  MATLAB Function2/1(alpha) -> MATLAB Function3/1(alpha)
  Constant1/1 -> Mod/2
  Sum2/1 -> Integrator/1
  MATLAB Function3/1(d) -> id/1
  Mod/1 -> MATLAB Function3/2(wt), MATLAB Function1/2(wt), Scope2/1, wt/1

== system MMC_Rectifier_NLM_2018/子模块投入个数 ==
  VA : Inport
  HLA : Inport  Port=2
  VB : Inport  Port=3
  HLB : Inport  Port=4
  VC : Inport  Port=5
  HLC : Inport  Port=6
  Subsystem : Subsystem
  Subsystem1 : Subsystem
  Subsystem2 : Subsystem
  Subsystem3 : Subsystem
  Subsystem4 : Subsystem
  Subsystem5 : Subsystem
  NAP : Outport
  NAL : Outport  Port=2
  NBP : Outport  Port=3
  NBL : Outport  Port=4
  NCP : Outport  Port=5
  NCL : Outport  Port=6
  wires:
  HLB/1 -> Subsystem3/2(HLB), Subsystem2/2(HLB)
  VB/1 -> Subsystem3/1(VB), Subsystem2/1(VB)
  HLA/1 -> Subsystem1/2(HLA), Subsystem/2(HLA)
  VC/1 -> Subsystem5/1(VC), Subsystem4/1(VC)
  VA/1 -> Subsystem1/1(VA), Subsystem/1(VA)
  Subsystem2/1(NBP) -> NBP/1
  HLC/1 -> Subsystem5/2(HLC), Subsystem4/2(HLC)
  Subsystem/1(NAP) -> NAP/1
  Subsystem3/1(NBL) -> NBL/1
  Subsystem5/1(NCL) -> NCL/1
  Subsystem1/1(NAL) -> NAL/1
  Subsystem4/1(NCP) -> NCP/1

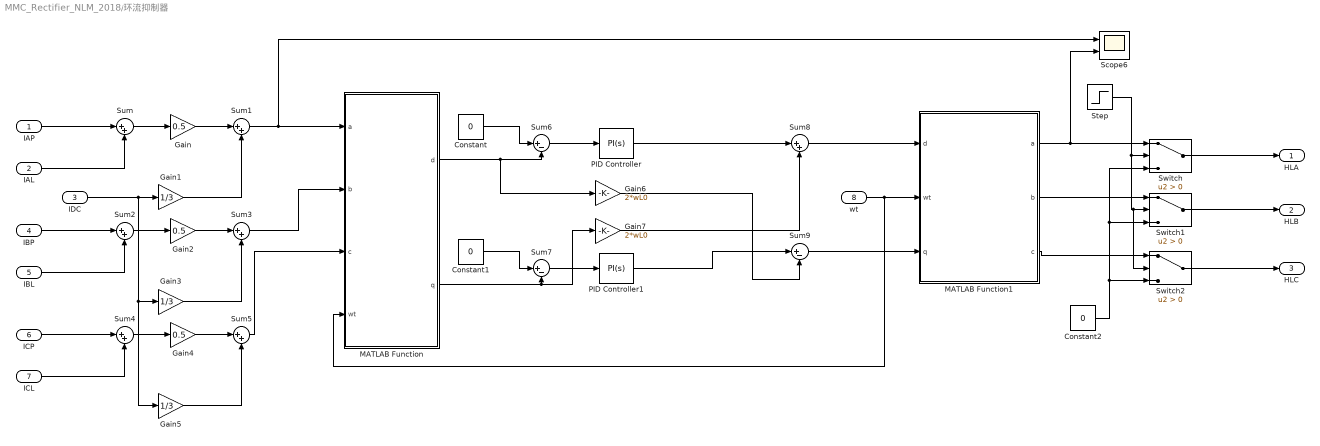
== system MMC_Rectifier_NLM_2018/环流抑制器 ==
  IAP : Inport
  IAL : Inport  Port=2
  IDC : Inport  Port=3
  IBP : Inport  Port=4
  IBL : Inport  Port=5
  ICP : Inport  Port=6
  ICL : Inport  Port=7
  wt : Inport  Port=8
  Constant : Constant  Value=0
  Constant1 : Constant  Value=0
  Constant2 : Constant  Value=0
  Gain : Gain  Gain=0.5
  Gain1 : Gain  Gain=1/3
  Gain2 : Gain  Gain=0.5
  Gain3 : Gain  Gain=1/3
  Gain4 : Gain  Gain=0.5
  Gain5 : Gain  Gain=1/3
  Gain6 : Gain  Gain=2*wL0
  Gain7 : Gain  Gain=2*wL0
  MATLAB Function : MATLAB Function  TreatAsAtomicUnit=on
  MATLAB Function1 : MATLAB Function  TreatAsAtomicUnit=on
  PID Controller : slpidlib/PID Controller  Controller=PI  Form=Parallel  TimeDomain=Continuous-time  UseExternalTs=off  SampleTime=-1  IntegratorMethod=Forward Euler  FilterMethod=Forward Euler  ControllerParametersSource=internal  P=KP  I=KI  UseKiTs=off  D=0  N=100  UseFilter=on  TunerSelectOption=Transfer Function Based (PID Tuner App)  InitialConditionSource=internal  InitialConditionForIntegrator=0  InitialConditionForFilter=0  DifferentiatorICPrevScaledInput=0  ExternalReset=none  TrackingMode=off  Kt=1  LimitOutput=off  SatLimitsSource=internal  UpperSaturationLimit=inf  LowerSaturationLimit=-inf  LinearizeAsGain=on  AntiWindupMode=none  Kb=1  LimitIntegrator=off  UpperIntegratorSaturationLimit=inf  LowerIntegratorSaturationLimit=-inf  POutMin=[]  POutMax=[]  IOutMin=[]  IOutMax=[]  DOutMin=[]  DOutMax=[]  NOutMin=[]  NOutMax=[]  SumOutMin=[]  SumOutMax=[]  SaturationOutMin=[]  SaturationOutMax=[]  PParamMin=[]  PParamMax=[]  IParamMin=[]  IParamMax=[]  DParamMin=[]  DParamMax=[]  NParamMin=[]  NParamMax=[]  KbParamMin=[]  KbParamMax=[]  KtParamMin=[]  KtParamMax=[]  KbOutMin=[]  KbOutMax=[]  KtOutMin=[]  KtOutMax=[]  IntegratorOutMin=[]  IntegratorOutMax=[]  FilterOutMin=[]  FilterOutMax=[]  SumI1OutMin=[]  SumI1OutMax=[]  SumI2OutMin=[]  SumI2OutMax=[]  SumI3OutMin=[]  SumI3OutMax=[]  SumI4OutMin=[]  SumI4OutMax=[]  SumDOutMin=[]  SumDOutMax=[]  DifferentiatorOutMin=[]  DifferentiatorOutMax=[]  FilterDiffOutCoefMin=[]  FilterDiffOutCoefMax=[]  ReciprocalOutMin=[]  ReciprocalOutMax=[]  SumDenOutMin=[]  SumDenOutMax=[]  SumNumOutMin=[]  SumNumOutMax=[]  DivideOutMin=[]  DivideOutMax=[]  UdiffTsProdOutMin=[]  UdiffTsProdOutMax=[]  NTsProdOutMin=[]  NTsProdOutMax=[]  UintegralTsProdOutMin=[]  UintegralTsProdOutMax=[]  UngainTsProdOutMin=[]  UngainTsProdOutMax=[]  ClampingZeroOutDataTypeStr=Inherit: Inherit via back propagation  ClampingZeroOutMin=[]  ClampingZeroOutMax=[]  FilterDenConstantOutDataTypeStr=Inherit: Inherit via back propagation  FilterDenConstantOutMin=[]  FilterDenConstantOutMax=[]  PCopyOutDataTypeStr=Inherit: Inherit via back propagation  PCopyOutMin=[]  PCopyOutMax=[]  NCopyOutDataTypeStr=Inherit: Inherit via back propagation  NCopyOutMin=[]  NCopyOutMax=[]  IntegratorContinuousStateAttributes=''  IntegratorStateMustResolveToSignalObject=off  IntegratorRTWStateStorageClass=Auto  FilterContinuousStateAttributes=''  FilterStateMustResolveToSignalObject=off  FilterRTWStateStorageClass=Auto  ParallelPVariant=InternalParameters  IdealPVariant=Disabled  IVariant=InternalParameters  DVariant=Disabled  IntegratorVariant=Continuous  SatVariant=Disabled  AWVariant=Passthrough  PCopyVariant=Disabled  TRVariant=Disabled  FdbkBlocksVariant=Forward  IdealPFdbkVariant=Disabled  SatFdbkVariant=Disabled  DerivativeFilterVariant=Disabled  NVariant=Disabled  NCopyVariant=Disabled_SignalSpec  FilterICVariant=Disabled  IntegratorICVariant=InternalICs  ExternalResetVariant=Disabled  TRSumVariant=Passthrough  SumFdbkVariant=Disabled  SumVariant=Sum_PI  TsampFilterVariant=InternalTs  TsampNgainVariant=Passthrough  TsampIntegralVariant=Disabled_SignalSpec  ExternalSaturationOutDataTypeStr=Inherit: Same as second input
  PID Controller1 : slpidlib/PID Controller  Controller=PI  Form=Parallel  TimeDomain=Continuous-time  UseExternalTs=off  SampleTime=-1  IntegratorMethod=Forward Euler  FilterMethod=Forward Euler  ControllerParametersSource=internal  P=KP  I=KI  UseKiTs=off  D=0  N=100  UseFilter=on  TunerSelectOption=Transfer Function Based (PID Tuner App)  InitialConditionSource=internal  InitialConditionForIntegrator=0  InitialConditionForFilter=0  DifferentiatorICPrevScaledInput=0  ExternalReset=none  TrackingMode=off  Kt=1  LimitOutput=off  SatLimitsSource=internal  UpperSaturationLimit=inf  LowerSaturationLimit=-inf  LinearizeAsGain=on  AntiWindupMode=none  Kb=1  LimitIntegrator=off  UpperIntegratorSaturationLimit=inf  LowerIntegratorSaturationLimit=-inf  POutMin=[]  POutMax=[]  IOutMin=[]  IOutMax=[]  DOutMin=[]  DOutMax=[]  NOutMin=[]  NOutMax=[]  SumOutMin=[]  SumOutMax=[]  SaturationOutMin=[]  SaturationOutMax=[]  PParamMin=[]  PParamMax=[]  IParamMin=[]  IParamMax=[]  DParamMin=[]  DParamMax=[]  NParamMin=[]  NParamMax=[]  KbParamMin=[]  KbParamMax=[]  KtParamMin=[]  KtParamMax=[]  KbOutMin=[]  KbOutMax=[]  KtOutMin=[]  KtOutMax=[]  IntegratorOutMin=[]  IntegratorOutMax=[]  FilterOutMin=[]  FilterOutMax=[]  SumI1OutMin=[]  SumI1OutMax=[]  SumI2OutMin=[]  SumI2OutMax=[]  SumI3OutMin=[]  SumI3OutMax=[]  SumI4OutMin=[]  SumI4OutMax=[]  SumDOutMin=[]  SumDOutMax=[]  DifferentiatorOutMin=[]  DifferentiatorOutMax=[]  FilterDiffOutCoefMin=[]  FilterDiffOutCoefMax=[]  ReciprocalOutMin=[]  ReciprocalOutMax=[]  SumDenOutMin=[]  SumDenOutMax=[]  SumNumOutMin=[]  SumNumOutMax=[]  DivideOutMin=[]  DivideOutMax=[]  UdiffTsProdOutMin=[]  UdiffTsProdOutMax=[]  NTsProdOutMin=[]  NTsProdOutMax=[]  UintegralTsProdOutMin=[]  UintegralTsProdOutMax=[]  UngainTsProdOutMin=[]  UngainTsProdOutMax=[]  ClampingZeroOutDataTypeStr=Inherit: Inherit via back propagation  ClampingZeroOutMin=[]  ClampingZeroOutMax=[]  FilterDenConstantOutDataTypeStr=Inherit: Inherit via back propagation  FilterDenConstantOutMin=[]  FilterDenConstantOutMax=[]  PCopyOutDataTypeStr=Inherit: Inherit via back propagation  PCopyOutMin=[]  PCopyOutMax=[]  NCopyOutDataTypeStr=Inherit: Inherit via back propagation  NCopyOutMin=[]  NCopyOutMax=[]  IntegratorContinuousStateAttributes=''  IntegratorStateMustResolveToSignalObject=off  IntegratorRTWStateStorageClass=Auto  FilterContinuousStateAttributes=''  FilterStateMustResolveToSignalObject=off  FilterRTWStateStorageClass=Auto  ParallelPVariant=InternalParameters  IdealPVariant=Disabled  IVariant=InternalParameters  DVariant=Disabled  IntegratorVariant=Continuous  SatVariant=Disabled  AWVariant=Passthrough  PCopyVariant=Disabled  TRVariant=Disabled  FdbkBlocksVariant=Forward  IdealPFdbkVariant=Disabled  SatFdbkVariant=Disabled  DerivativeFilterVariant=Disabled  NVariant=Disabled  NCopyVariant=Disabled_SignalSpec  FilterICVariant=Disabled  IntegratorICVariant=InternalICs  ExternalResetVariant=Disabled  TRSumVariant=Passthrough  SumFdbkVariant=Disabled  SumVariant=Sum_PI  TsampFilterVariant=InternalTs  TsampNgainVariant=Passthrough  TsampIntegralVariant=Disabled_SignalSpec  ExternalSaturationOutDataTypeStr=Inherit: Same as second input
  Scope6 : Scope  NumInputPorts=2
  Step : Step  Time=1.5  SampleTime=0
  Sum{,1..5,8} (7 alike) : Sum  Inputs=|++
  Sum6 : Sum  Inputs=|+-
  Sum7 : Sum  Inputs=|+-
  Sum9 : Sum  Inputs=|+-
  Switch : Switch  Criteria=u2 > Threshold  SaturateOnIntegerOverflow=off  InputSameDT=off
  Switch1 : Switch  Criteria=u2 > Threshold  SaturateOnIntegerOverflow=off  InputSameDT=off
  Switch2 : Switch  Criteria=u2 > Threshold  SaturateOnIntegerOverflow=off  InputSameDT=off
  HLA : Outport
  HLB : Outport  Port=2
  HLC : Outport  Port=3
  wires:
  Gain1/1 -> Sum1/2
  Sum3/1 -> MATLAB Function/2(b)
  Constant/1 -> Sum6/1
  IAP/1 -> Sum/1
  Sum2/1 -> Gain2/1
  ICL/1 -> Sum4/2
  Switch/1 -> HLA/1
  Constant2/1 -> Switch2/3, Switch1/3, Switch/3
  Step/1 -> Switch2/2, Switch1/2, Switch/2
  IBP/1 -> Sum2/1
  Sum/1 -> Gain/1
  Sum6/1 -> PID Controller/1
  Gain/1 -> Sum1/1
  IAL/1 -> Sum/2
  MATLAB Function/1(d) -> Gain6/1, Sum6/2
  Sum1/1 -> Scope6/1, MATLAB Function/1(a)
  MATLAB Function/2(q) -> Gain7/1, Sum7/2
  IDC/1 -> Gain5/1, Gain3/1, Gain1/1
  MATLAB Function1/1(a) -> Scope6/2, Switch/1
  Sum5/1 -> MATLAB Function/3(c)
  MATLAB Function1/2(b) -> Switch1/1
  Gain3/1 -> Sum3/2
  ICP/1 -> Sum4/1
  Sum4/1 -> Gain4/1
  wt/1 -> MATLAB Function/4(wt), MATLAB Function1/2(wt)
  Switch1/1 -> HLB/1
  Gain2/1 -> Sum3/1
  Switch2/1 -> HLC/1
  IBL/1 -> Sum2/2
  Gain4/1 -> Sum5/1
  Gain5/1 -> Sum5/2
  PID Controller/1 -> Sum8/1
  MATLAB Function1/3(c) -> Switch2/1
  Sum7/1 -> PID Controller1/1
  Constant1/1 -> Sum7/1
  Gain7/1 -> Sum8/2
  Sum8/1 -> MATLAB Function1/1(d)
  Sum9/1 -> MATLAB Function1/3(q)
  PID Controller1/1 -> Sum9/1
  Gain6/1 -> Sum9/2

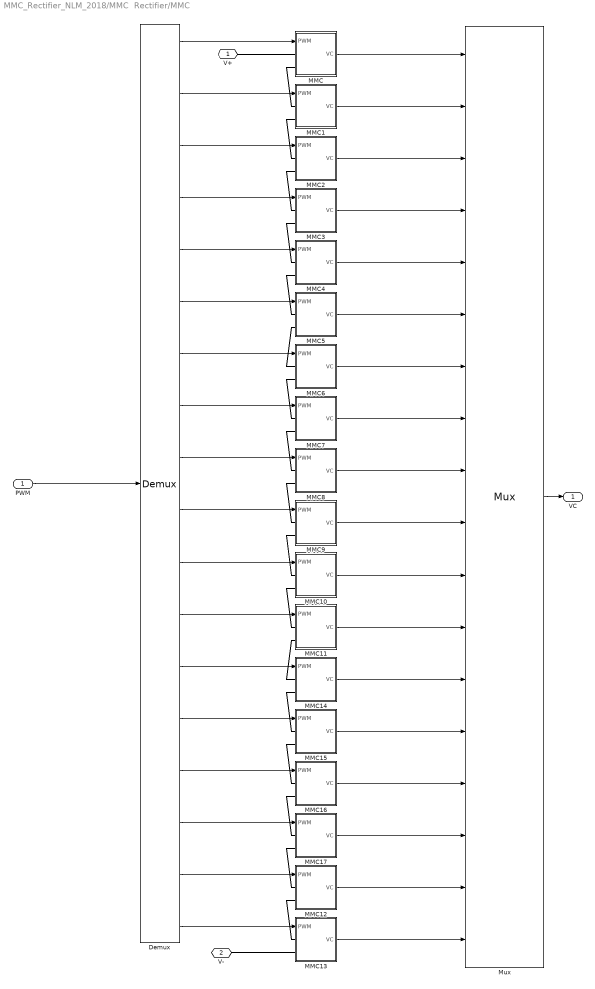
== system MMC_Rectifier_NLM_2018/MMC  Rectifier/MMC ==
  PWM : Inport
  Demux : Demux  Outputs=18
  MMC : Subsystem
  MMC1 : Subsystem
  MMC10 : Subsystem
  MMC11 : Subsystem
  MMC12 : Subsystem
  MMC13 : Subsystem
  MMC14 : Subsystem
  MMC15 : Subsystem
  MMC16 : Subsystem
  MMC17 : Subsystem
  MMC2 : Subsystem
  MMC3 : Subsystem
  MMC4 : Subsystem
  MMC5 : Subsystem
  MMC6 : Subsystem
  MMC7 : Subsystem
  MMC8 : Subsystem
  MMC9 : Subsystem
  Mux : Mux  Inputs=18
  V+ : PMIOPort  Side=Left
  V- : PMIOPort  Port=2  Side=Left
  VC : Outport
  wires:
  MMC/1(VC) -> Mux/1
  MMC1/1(VC) -> Mux/2
  MMC2/1(VC) -> Mux/3
  MMC3/1(VC) -> Mux/4
  MMC4/1(VC) -> Mux/5
  MMC5/1(VC) -> Mux/6
  MMC6/1(VC) -> Mux/7
  MMC7/1(VC) -> Mux/8
  MMC8/1(VC) -> Mux/9
  MMC9/1(VC) -> Mux/10
  MMC10/1(VC) -> Mux/11
  MMC11/1(VC) -> Mux/12
  MMC14/1(VC) -> Mux/13
  MMC15/1(VC) -> Mux/14
  MMC16/1(VC) -> Mux/15
  MMC17/1(VC) -> Mux/16
  MMC12/1(VC) -> Mux/17
  MMC13/1(VC) -> Mux/18
  Mux/1 -> VC/1
  Demux/1 -> MMC/1(PWM)
  Demux/2 -> MMC1/1(PWM)
  Demux/3 -> MMC2/1(PWM)
  Demux/4 -> MMC3/1(PWM)
  Demux/5 -> MMC4/1(PWM)
  Demux/6 -> MMC5/1(PWM)
  Demux/7 -> MMC6/1(PWM)
  Demux/8 -> MMC7/1(PWM)
  Demux/9 -> MMC8/1(PWM)
  Demux/10 -> MMC9/1(PWM)
  Demux/11 -> MMC10/1(PWM)
  Demux/12 -> MMC11/1(PWM)
  Demux/13 -> MMC14/1(PWM)
  Demux/14 -> MMC15/1(PWM)
  Demux/15 -> MMC16/1(PWM)
  Demux/16 -> MMC17/1(PWM)
  Demux/17 -> MMC12/1(PWM)
  Demux/18 -> MMC13/1(PWM)
  PWM/1 -> Demux/1
  connections:
  MMC4/LConn2 -- MMC5/LConn1
  MMC/LConn2 -- MMC1/LConn1
  MMC1/LConn2 -- MMC2/LConn1
  MMC2/LConn2 -- MMC3/LConn1
  MMC3/LConn2 -- MMC4/LConn1
  MMC9/LConn2 -- MMC10/LConn1
  MMC8/LConn2 -- MMC9/LConn1
  MMC7/LConn2 -- MMC8/LConn1
  MMC6/LConn2 -- MMC7/LConn1
  MMC10/LConn2 -- MMC11/LConn1
  MMC12/LConn2 -- MMC13/LConn1
  MMC14/LConn2 -- MMC15/LConn1
  MMC16/LConn2 -- MMC17/LConn1
  MMC17/LConn2 -- MMC12/LConn1
  MMC15/LConn2 -- MMC16/LConn1
  MMC14/LConn1 -- MMC11/LConn2
  MMC6/LConn1 -- MMC5/LConn2
  V-/RConn1 -- MMC13/LConn2
  V+/RConn1 -- MMC/LConn1

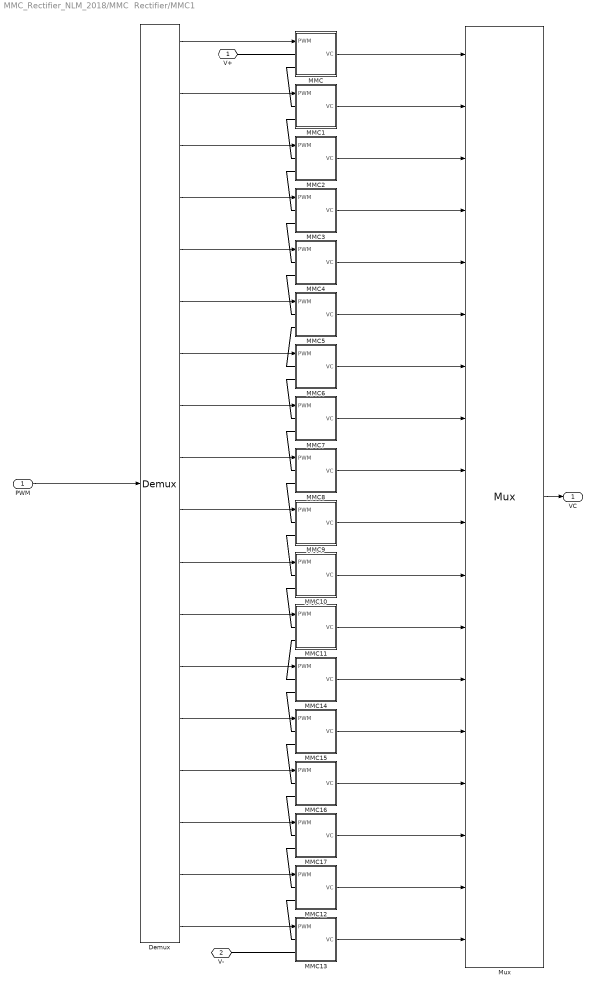
== system MMC_Rectifier_NLM_2018/MMC  Rectifier/MMC1 ==
  PWM : Inport
  Demux : Demux  Outputs=18
  MMC : Subsystem
  MMC1 : Subsystem
  MMC10 : Subsystem
  MMC11 : Subsystem
  MMC12 : Subsystem
  MMC13 : Subsystem
  MMC14 : Subsystem
  MMC15 : Subsystem
  MMC16 : Subsystem
  MMC17 : Subsystem
  MMC2 : Subsystem
  MMC3 : Subsystem
  MMC4 : Subsystem
  MMC5 : Subsystem
  MMC6 : Subsystem
  MMC7 : Subsystem
  MMC8 : Subsystem
  MMC9 : Subsystem
  Mux : Mux  Inputs=18
  V+ : PMIOPort  Side=Left
  V- : PMIOPort  Port=2  Side=Left
  VC : Outport
  wires:
  PWM/1 -> Demux/1
  Demux/18 -> MMC13/1(PWM)
  Demux/17 -> MMC12/1(PWM)
  Demux/16 -> MMC17/1(PWM)
  Demux/15 -> MMC16/1(PWM)
  Demux/14 -> MMC15/1(PWM)
  Demux/13 -> MMC14/1(PWM)
  Demux/12 -> MMC11/1(PWM)
  Demux/11 -> MMC10/1(PWM)
  Demux/10 -> MMC9/1(PWM)
  Demux/9 -> MMC8/1(PWM)
  Demux/8 -> MMC7/1(PWM)
  Demux/7 -> MMC6/1(PWM)
  Demux/6 -> MMC5/1(PWM)
  Demux/5 -> MMC4/1(PWM)
  Demux/4 -> MMC3/1(PWM)
  Demux/3 -> MMC2/1(PWM)
  Demux/2 -> MMC1/1(PWM)
  Demux/1 -> MMC/1(PWM)
  Mux/1 -> VC/1
  MMC13/1(VC) -> Mux/18
  MMC12/1(VC) -> Mux/17
  MMC17/1(VC) -> Mux/16
  MMC16/1(VC) -> Mux/15
  MMC15/1(VC) -> Mux/14
  MMC14/1(VC) -> Mux/13
  MMC11/1(VC) -> Mux/12
  MMC10/1(VC) -> Mux/11
  MMC9/1(VC) -> Mux/10
  MMC8/1(VC) -> Mux/9
  MMC7/1(VC) -> Mux/8
  MMC6/1(VC) -> Mux/7
  MMC5/1(VC) -> Mux/6
  MMC4/1(VC) -> Mux/5
  MMC3/1(VC) -> Mux/4
  MMC2/1(VC) -> Mux/3
  MMC1/1(VC) -> Mux/2
  MMC/1(VC) -> Mux/1
  connections:
  V+/RConn1 -- MMC/LConn1
  V-/RConn1 -- MMC13/LConn2
  MMC6/LConn1 -- MMC5/LConn2
  MMC14/LConn1 -- MMC11/LConn2
  MMC15/LConn2 -- MMC16/LConn1
  MMC17/LConn2 -- MMC12/LConn1
  MMC16/LConn2 -- MMC17/LConn1
  MMC14/LConn2 -- MMC15/LConn1
  MMC12/LConn2 -- MMC13/LConn1
  MMC10/LConn2 -- MMC11/LConn1
  MMC6/LConn2 -- MMC7/LConn1
  MMC7/LConn2 -- MMC8/LConn1
  MMC8/LConn2 -- MMC9/LConn1
  MMC9/LConn2 -- MMC10/LConn1
  MMC3/LConn2 -- MMC4/LConn1
  MMC2/LConn2 -- MMC3/LConn1
  MMC1/LConn2 -- MMC2/LConn1
  MMC/LConn2 -- MMC1/LConn1
  MMC4/LConn2 -- MMC5/LConn1

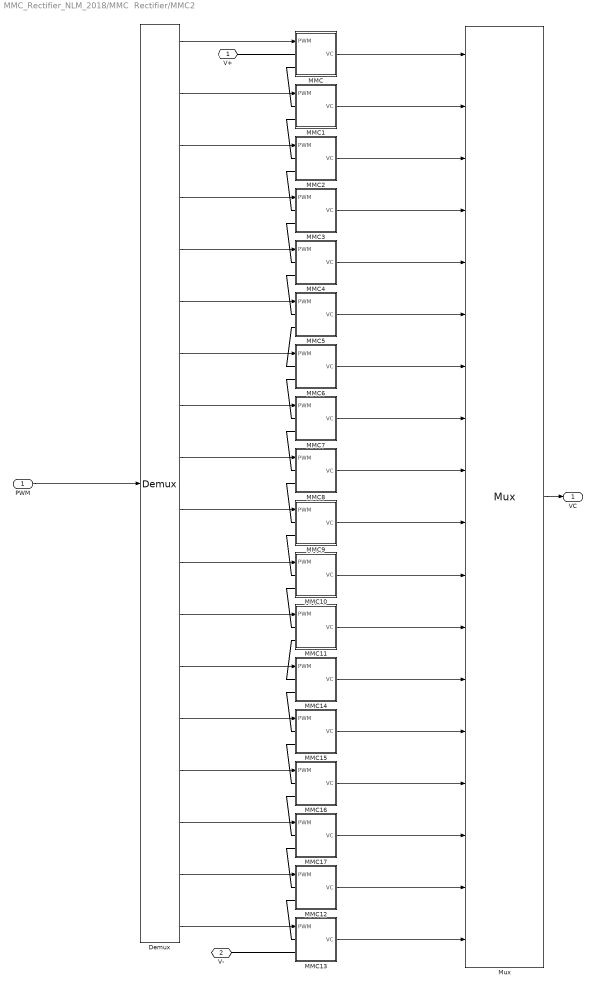
== system MMC_Rectifier_NLM_2018/MMC  Rectifier/MMC2 ==
  PWM : Inport
  Demux : Demux  Outputs=18
  MMC : Subsystem
  MMC1 : Subsystem
  MMC10 : Subsystem
  MMC11 : Subsystem
  MMC12 : Subsystem
  MMC13 : Subsystem
  MMC14 : Subsystem
  MMC15 : Subsystem
  MMC16 : Subsystem
  MMC17 : Subsystem
  MMC2 : Subsystem
  MMC3 : Subsystem
  MMC4 : Subsystem
  MMC5 : Subsystem
  MMC6 : Subsystem
  MMC7 : Subsystem
  MMC8 : Subsystem
  MMC9 : Subsystem
  Mux : Mux  Inputs=18
  V+ : PMIOPort  Side=Left
  V- : PMIOPort  Port=2  Side=Left
  VC : Outport
  wires:
  MMC/1(VC) -> Mux/1
  MMC1/1(VC) -> Mux/2
  MMC2/1(VC) -> Mux/3
  MMC3/1(VC) -> Mux/4
  MMC4/1(VC) -> Mux/5
  MMC5/1(VC) -> Mux/6
  MMC6/1(VC) -> Mux/7
  MMC7/1(VC) -> Mux/8
  MMC8/1(VC) -> Mux/9
  MMC9/1(VC) -> Mux/10
  MMC10/1(VC) -> Mux/11
  MMC11/1(VC) -> Mux/12
  MMC14/1(VC) -> Mux/13
  MMC15/1(VC) -> Mux/14
  MMC16/1(VC) -> Mux/15
  MMC17/1(VC) -> Mux/16
  MMC12/1(VC) -> Mux/17
  MMC13/1(VC) -> Mux/18
  Mux/1 -> VC/1
  Demux/1 -> MMC/1(PWM)
  Demux/2 -> MMC1/1(PWM)
  Demux/3 -> MMC2/1(PWM)
  Demux/4 -> MMC3/1(PWM)
  Demux/5 -> MMC4/1(PWM)
  Demux/6 -> MMC5/1(PWM)
  Demux/7 -> MMC6/1(PWM)
  Demux/8 -> MMC7/1(PWM)
  Demux/9 -> MMC8/1(PWM)
  Demux/10 -> MMC9/1(PWM)
  Demux/11 -> MMC10/1(PWM)
  Demux/12 -> MMC11/1(PWM)
  Demux/13 -> MMC14/1(PWM)
  Demux/14 -> MMC15/1(PWM)
  Demux/15 -> MMC16/1(PWM)
  Demux/16 -> MMC17/1(PWM)
  Demux/17 -> MMC12/1(PWM)
  Demux/18 -> MMC13/1(PWM)
  PWM/1 -> Demux/1
  connections:
  MMC4/LConn2 -- MMC5/LConn1
  MMC/LConn2 -- MMC1/LConn1
  MMC1/LConn2 -- MMC2/LConn1
  MMC2/LConn2 -- MMC3/LConn1
  MMC3/LConn2 -- MMC4/LConn1
  MMC9/LConn2 -- MMC10/LConn1
  MMC8/LConn2 -- MMC9/LConn1
  MMC7/LConn2 -- MMC8/LConn1
  MMC6/LConn2 -- MMC7/LConn1
  MMC10/LConn2 -- MMC11/LConn1
  MMC12/LConn2 -- MMC13/LConn1
  MMC14/LConn2 -- MMC15/LConn1
  MMC16/LConn2 -- MMC17/LConn1
  MMC17/LConn2 -- MMC12/LConn1
  MMC15/LConn2 -- MMC16/LConn1
  MMC14/LConn1 -- MMC11/LConn2
  MMC6/LConn1 -- MMC5/LConn2
  V-/RConn1 -- MMC13/LConn2
  V+/RConn1 -- MMC/LConn1

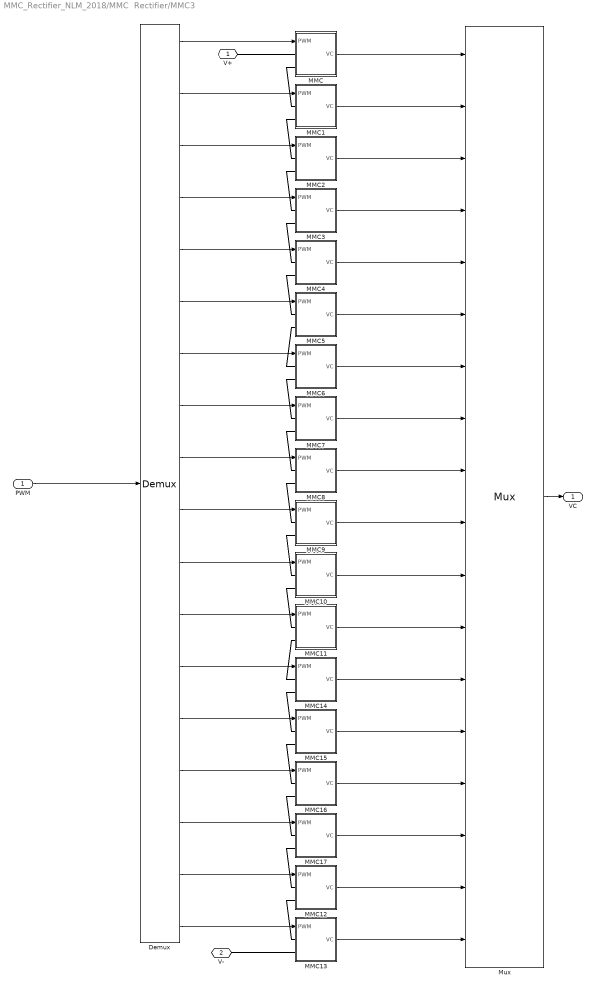
== system MMC_Rectifier_NLM_2018/MMC  Rectifier/MMC3 ==
  PWM : Inport
  Demux : Demux  Outputs=18
  MMC : Subsystem
  MMC1 : Subsystem
  MMC10 : Subsystem
  MMC11 : Subsystem
  MMC12 : Subsystem
  MMC13 : Subsystem
  MMC14 : Subsystem
  MMC15 : Subsystem
  MMC16 : Subsystem
  MMC17 : Subsystem
  MMC2 : Subsystem
  MMC3 : Subsystem
  MMC4 : Subsystem
  MMC5 : Subsystem
  MMC6 : Subsystem
  MMC7 : Subsystem
  MMC8 : Subsystem
  MMC9 : Subsystem
  Mux : Mux  Inputs=18
  V+ : PMIOPort  Side=Left
  V- : PMIOPort  Port=2  Side=Left
  VC : Outport
  wires:
  PWM/1 -> Demux/1
  Demux/18 -> MMC13/1(PWM)
  Demux/17 -> MMC12/1(PWM)
  Demux/16 -> MMC17/1(PWM)
  Demux/15 -> MMC16/1(PWM)
  Demux/14 -> MMC15/1(PWM)
  Demux/13 -> MMC14/1(PWM)
  Demux/12 -> MMC11/1(PWM)
  Demux/11 -> MMC10/1(PWM)
  Demux/10 -> MMC9/1(PWM)
  Demux/9 -> MMC8/1(PWM)
  Demux/8 -> MMC7/1(PWM)
  Demux/7 -> MMC6/1(PWM)
  Demux/6 -> MMC5/1(PWM)
  Demux/5 -> MMC4/1(PWM)
  Demux/4 -> MMC3/1(PWM)
  Demux/3 -> MMC2/1(PWM)
  Demux/2 -> MMC1/1(PWM)
  Demux/1 -> MMC/1(PWM)
  Mux/1 -> VC/1
  MMC13/1(VC) -> Mux/18
  MMC12/1(VC) -> Mux/17
  MMC17/1(VC) -> Mux/16
  MMC16/1(VC) -> Mux/15
  MMC15/1(VC) -> Mux/14
  MMC14/1(VC) -> Mux/13
  MMC11/1(VC) -> Mux/12
  MMC10/1(VC) -> Mux/11
  MMC9/1(VC) -> Mux/10
  MMC8/1(VC) -> Mux/9
  MMC7/1(VC) -> Mux/8
  MMC6/1(VC) -> Mux/7
  MMC5/1(VC) -> Mux/6
  MMC4/1(VC) -> Mux/5
  MMC3/1(VC) -> Mux/4
  MMC2/1(VC) -> Mux/3
  MMC1/1(VC) -> Mux/2
  MMC/1(VC) -> Mux/1
  connections:
  V+/RConn1 -- MMC/LConn1
  V-/RConn1 -- MMC13/LConn2
  MMC6/LConn1 -- MMC5/LConn2
  MMC14/LConn1 -- MMC11/LConn2
  MMC15/LConn2 -- MMC16/LConn1
  MMC17/LConn2 -- MMC12/LConn1
  MMC16/LConn2 -- MMC17/LConn1
  MMC14/LConn2 -- MMC15/LConn1
  MMC12/LConn2 -- MMC13/LConn1
  MMC10/LConn2 -- MMC11/LConn1
  MMC6/LConn2 -- MMC7/LConn1
  MMC7/LConn2 -- MMC8/LConn1
  MMC8/LConn2 -- MMC9/LConn1
  MMC9/LConn2 -- MMC10/LConn1
  MMC3/LConn2 -- MMC4/LConn1
  MMC2/LConn2 -- MMC3/LConn1
  MMC1/LConn2 -- MMC2/LConn1
  MMC/LConn2 -- MMC1/LConn1
  MMC4/LConn2 -- MMC5/LConn1

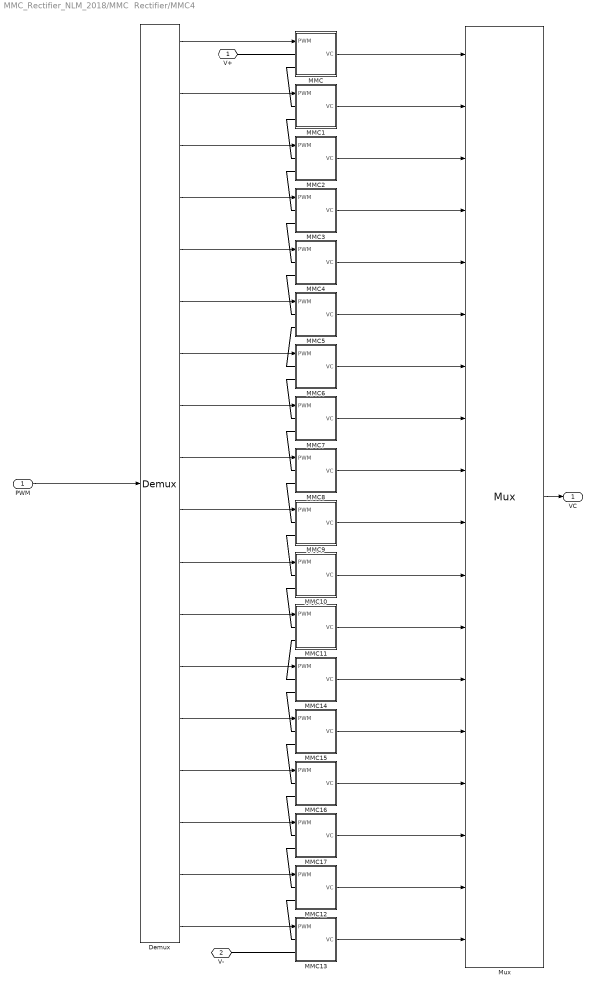
== system MMC_Rectifier_NLM_2018/MMC  Rectifier/MMC4 ==
  PWM : Inport
  Demux : Demux  Outputs=18
  MMC : Subsystem
  MMC1 : Subsystem
  MMC10 : Subsystem
  MMC11 : Subsystem
  MMC12 : Subsystem
  MMC13 : Subsystem
  MMC14 : Subsystem
  MMC15 : Subsystem
  MMC16 : Subsystem
  MMC17 : Subsystem
  MMC2 : Subsystem
  MMC3 : Subsystem
  MMC4 : Subsystem
  MMC5 : Subsystem
  MMC6 : Subsystem
  MMC7 : Subsystem
  MMC8 : Subsystem
  MMC9 : Subsystem
  Mux : Mux  Inputs=18
  V+ : PMIOPort  Side=Left
  V- : PMIOPort  Port=2  Side=Left
  VC : Outport
  wires:
  MMC/1(VC) -> Mux/1
  MMC1/1(VC) -> Mux/2
  MMC2/1(VC) -> Mux/3
  MMC3/1(VC) -> Mux/4
  MMC4/1(VC) -> Mux/5
  MMC5/1(VC) -> Mux/6
  MMC6/1(VC) -> Mux/7
  MMC7/1(VC) -> Mux/8
  MMC8/1(VC) -> Mux/9
  MMC9/1(VC) -> Mux/10
  MMC10/1(VC) -> Mux/11
  MMC11/1(VC) -> Mux/12
  MMC14/1(VC) -> Mux/13
  MMC15/1(VC) -> Mux/14
  MMC16/1(VC) -> Mux/15
  MMC17/1(VC) -> Mux/16
  MMC12/1(VC) -> Mux/17
  MMC13/1(VC) -> Mux/18
  Mux/1 -> VC/1
  Demux/1 -> MMC/1(PWM)
  Demux/2 -> MMC1/1(PWM)
  Demux/3 -> MMC2/1(PWM)
  Demux/4 -> MMC3/1(PWM)
  Demux/5 -> MMC4/1(PWM)
  Demux/6 -> MMC5/1(PWM)
  Demux/7 -> MMC6/1(PWM)
  Demux/8 -> MMC7/1(PWM)
  Demux/9 -> MMC8/1(PWM)
  Demux/10 -> MMC9/1(PWM)
  Demux/11 -> MMC10/1(PWM)
  Demux/12 -> MMC11/1(PWM)
  Demux/13 -> MMC14/1(PWM)
  Demux/14 -> MMC15/1(PWM)
  Demux/15 -> MMC16/1(PWM)
  Demux/16 -> MMC17/1(PWM)
  Demux/17 -> MMC12/1(PWM)
  Demux/18 -> MMC13/1(PWM)
  PWM/1 -> Demux/1
  connections:
  MMC4/LConn2 -- MMC5/LConn1
  MMC/LConn2 -- MMC1/LConn1
  MMC1/LConn2 -- MMC2/LConn1
  MMC2/LConn2 -- MMC3/LConn1
  MMC3/LConn2 -- MMC4/LConn1
  MMC9/LConn2 -- MMC10/LConn1
  MMC8/LConn2 -- MMC9/LConn1
  MMC7/LConn2 -- MMC8/LConn1
  MMC6/LConn2 -- MMC7/LConn1
  MMC10/LConn2 -- MMC11/LConn1
  MMC12/LConn2 -- MMC13/LConn1
  MMC14/LConn2 -- MMC15/LConn1
  MMC16/LConn2 -- MMC17/LConn1
  MMC17/LConn2 -- MMC12/LConn1
  MMC15/LConn2 -- MMC16/LConn1
  MMC14/LConn1 -- MMC11/LConn2
  MMC6/LConn1 -- MMC5/LConn2
  V-/RConn1 -- MMC13/LConn2
  V+/RConn1 -- MMC/LConn1
